simulink model "gnc_LocalAvoidance"  (R2026b)
settings: Solver=VariableStepAuto
values from neighbouring files (symbols this model uses):
  D = min(D, hypot(X - px(q) - t*ux, Y - py(q) - t*uy))    [gnc_globalReplanner.m]    (also in gnc_mpcPlantUpdate.m = zeros(2, 5))
  Ts = prm.Ts    [gnc_missionFSM.m]    (also in gnc_mpcPlantUpdate.m)
undefined symbols (not defined in the file or in its folder): P
libraries: simulink x3, navlib x1, robotalgslib x1
settings Model: Creator=aomar  LastModifiedBy=aomar

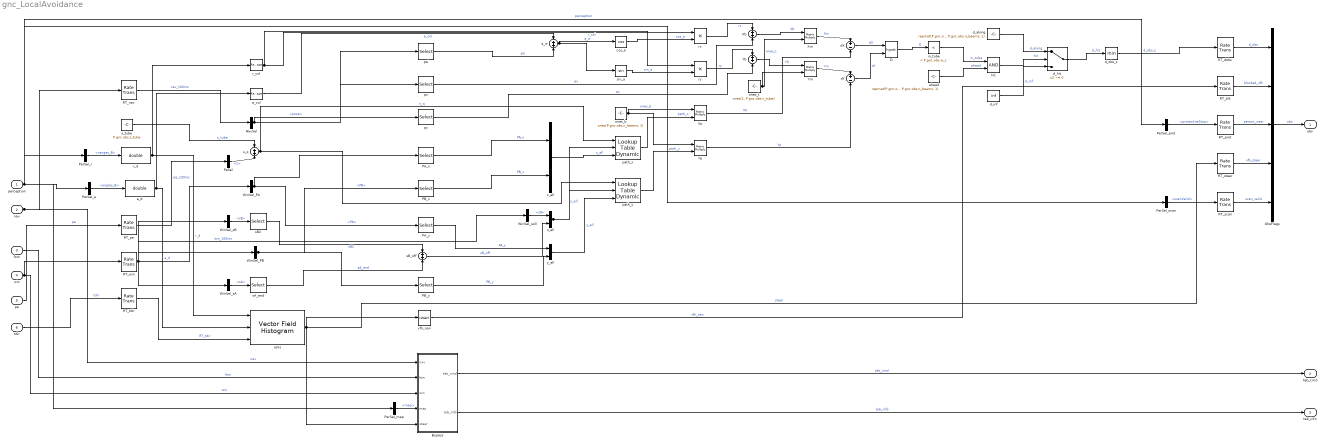
== system gnc_LocalAvoidance ==
  perception : Inport  OutDataTypeStr=Bus: Bus_Perception  SampleTime=Ts.perception
  nav : Inport  Port=2  OutDataTypeStr=Bus: Bus_NavCond  SampleTime=Ts.gnc
  fsm : Inport  Port=3  OutDataTypeStr=Bus: Bus_FsmOut  SampleTime=Ts.gnc
  win : Inport  Port=4  OutDataTypeStr=Bus: Bus_PathWindow  SampleTime=Ts.gnc
  pe : Inport  Port=5  OutDataTypeStr=Bus: Bus_PathError  SampleTime=Ts.gnc
  tdir : Inport  Port=6  OutDataTypeStr=double  PortDimensions=1  SampleTime=Ts.gnc
  Bypass : Subsystem  Variant=on
  D : Math  Operator=hypot
  NavSel : BusSelector  OutputSignals=pose
  ObsFlags : BusCreator  Inputs=5  OutDataTypeStr=Bus: Bus_ObsFlags  NonVirtualBus=on
  PA_x : Selector  NumberOfDimensions=2  InputPortWidth=3  IndexOptions=Select all,Index vector (dialog)  Indices=,1  OutputSizes=1
  PA_y : Selector  NumberOfDimensions=2  InputPortWidth=3  IndexOptions=Select all,Index vector (dialog)  Indices=,2  OutputSizes=1
  PB_x : Selector  NumberOfDimensions=2  InputPortWidth=3  IndexOptions=Index vector (dialog),Index vector (dialog)  Indices=2:P.gnc.path.N_smooth,1  OutputSizes=1
  PB_y : Selector  NumberOfDimensions=2  InputPortWidth=3  IndexOptions=Index vector (dialog),Index vector (dialog)  Indices=2:P.gnc.path.N_smooth,2  OutputSizes=1
  PeSel : BusSelector  OutputSignals=s
  PerSel_a : BusSelector  OutputSignals=angles_B
  PerSel_map : BusSelector  OutputSignals=map
  PerSel_prot : BusSelector  OutputSignals=protectiveStop
  PerSel_r : BusSelector  OutputSignals=ranges_B
  PerSel_scan : BusSelector  OutputSignals=scanValid
  RT_blk : RateTransition  OutPortSampleTime=Ts.gnc
  RT_dobs : RateTransition  InitialCondition=1e6  OutPortSampleTime=Ts.gnc
  RT_nav : RateTransition  OutPortSampleTime=Ts.gnc_avoid
  RT_pe : RateTransition  OutPortSampleTime=Ts.gnc_avoid
  RT_prot : RateTransition  OutPortSampleTime=Ts.gnc
  RT_scan : RateTransition  InitialCondition=false  OutPortSampleTime=Ts.gnc
  RT_steer : RateTransition  OutPortSampleTime=Ts.gnc
  RT_tdir : RateTransition  OutPortSampleTime=Ts.gnc_avoid
  RT_win : RateTransition  OutPortSampleTime=Ts.gnc_avoid
  VFH : robotalgslib/Vector Field Histogram  NumAngularSectors=P.gnc.vfh.NumAngularSectors  DistanceLimits=P.gnc.vfh.DistanceLimits  HistogramThresholds=P.gnc.vfh.HistogramThresholds  RobotRadius=P.gnc.vfh.RobotRadius  SafetyDistance=P.gnc.vfh.SafetyDistance  MinTurningRadius=P.gnc.vfh.MinTurningRadius  SimulateUsing=Code generation  TargetDirectionWeight=P.gnc.vfh.TargetDirectionWeight  CurrentDirectionWeight=P.gnc.vfh.CurrentDirectionWeight  PreviousDirectionWeight=P.gnc.vfh.PreviousDirectionWeight
      settings: LibrarySourceBlock=navlib/Control Algorithms/Vector Field Histogram
  WinSel_PA : BusSelector  OutputSignals=PA
  WinSel_PB : BusSelector  OutputSignals=PB
  WinSel_sA : BusSelector  OutputSignals=sA
  WinSel_sAll : BusSelector  OutputSignals=sA
  WinSel_sB : BusSelector  OutputSignals=sB
  Xb : Sum
  Xm : Product  Inputs=**  Multiplication=Matrix(*)
  Xp : Product  Inputs=**  Multiplication=Matrix(*)
  Yb : Sum
  Ym : Product  Inputs=**  Multiplication=Matrix(*)
  Yp : Product  Inputs=**  Multiplication=Matrix(*)
  a_col : Reshape  OutputDimensionality=Column vector (2-D)
  a_d : DataTypeConversion  OutDataTypeStr=double  RndMeth=Nearest
  a_w : Sum
  ahead : Constant  Value=repmat(P.gnc.obs.s_tube > P.gnc.obs.x_f, P.gnc.obs.n_beams, 1)  OutDataTypeStr=boolean  SampleTime=Ts.gnc_avoid
  cos_a : Trigonometry  Operator=cos
  dX : Sum  Inputs=+-
  dY : Sum  Inputs=+-
  d_along : Constant  Value=repmat(P.gnc.obs.s_tube - P.gnc.obs.x_f, P.gnc.obs.n_beams, 1)  OutDataTypeStr=double  SampleTime=Ts.gnc_avoid
  d_hit : Switch  Criteria=u2 ~= 0  SaturateOnIntegerOverflow=off  InputSameDT=off
  d_inf : Constant  Value=inf  OutDataTypeStr=double  SampleTime=Ts.gnc_avoid
  d_obs_s : MinMax
  hit : Logic  AllPortsSameDT=off  OutDataTypeStr=boolean
  in_tube : simulink/Logic and Bit Operations/Compare To Constant  relop=<  const=P.gnc.obs.w_c  OutDataTypeStr=boolean
  ones_b : Constant  Value=ones(P.gnc.obs.n_beams, 1)  VectorParams1D=off  OutDataTypeStr=double  SampleTime=Ts.gnc_avoid
  ones_t : Constant  Value=ones(1, P.gnc.obs.n_tube)  VectorParams1D=off  OutDataTypeStr=double  SampleTime=Ts.gnc_avoid
  path_x : simulink/Lookup Tables/Lookup Table Dynamic  LookUpMeth=Interpolation-Use End Values  OutDataType=fixdt('double')  OutScaling=2^-10  OutputDataTypeScalingMode=Specify via dialog  OutDataTypeStr=double  DoSatur=off
  path_y : simulink/Lookup Tables/Lookup Table Dynamic  LookUpMeth=Interpolation-Use End Values  OutDataType=fixdt('double')  OutScaling=2^-10  OutputDataTypeScalingMode=Specify via dialog  OutDataTypeStr=double  DoSatur=off
  psi : Selector  IndexOptions=Index vector (dialog)  Indices=3  OutputSizes=1
  px : Selector  IndexOptions=Index vector (dialog)  Indices=1  OutputSizes=1
  py : Selector  IndexOptions=Index vector (dialog)  Indices=2  OutputSizes=1
  r_col : Reshape  OutputDimensionality=Column vector (2-D)
  r_d : DataTypeConversion  OutDataTypeStr=double  RndMeth=Nearest
  rx : Product  Inputs=**
  ry : Product  Inputs=**
  sA_end : Selector  IndexOptions=Index vector (dialog)  Indices=P.gnc.path.N_smooth  OutputSizes=1
  sB2 : Selector  IndexOptions=Index vector (dialog)  Indices=2:P.gnc.path.N_smooth  OutputSizes=1
  sB_off : Sum
  s_all : Concatenate
  s_q : Sum
  s_tube : Constant  Value=P.gnc.obs.s_tube  VectorParams1D=off  OutDataTypeStr=double  SampleTime=Ts.gnc_avoid
  sin_a : Trigonometry
  vfh_nan : RelationalOperator  Operator=isNaN  OutDataTypeStr=boolean  RndMeth=Simplest  InputSameDT=off
  x_all : Concatenate
  y_all : Concatenate
  obs : Outport  OutDataTypeStr=Bus: Bus_ObsFlags
  teb_cmd : Outport  Port=2  OutDataTypeStr=double
  teb_info : Outport  Port=3  OutDataTypeStr=double
  wires:
  perception/1 -> PerSel_map/1, PerSel_prot/1, PerSel_r/1, PerSel_scan/1, PerSel_a/1  "perception"
  nav/1 -> Bypass/1(nav), RT_nav/1  "nav"
  fsm/1 -> Bypass/2(fsm)  "fsm"
  win/1 -> Bypass/3(win), RT_win/1  "win"
  pe/1 -> RT_pe/1  "pe"
  tdir/1 -> RT_tdir/1  "tdir"
  PerSel_r/1 -> r_d/1  "<ranges_B>"
  PerSel_a/1 -> a_d/1  "<angles_B>"
  s_tube/1 -> s_q/1  "s_tube"
  RT_nav/1 -> NavSel/1  "nav_100ms"
  RT_pe/1 -> PeSel/1  "pe_100ms"
  RT_win/1 -> WinSel_PA/1, WinSel_sAll/1, WinSel_sB/1, WinSel_sA/1, WinSel_PB/1  "win_100ms"
  RT_tdir/1 -> VFH/3  "RT_tdir"
  r_d/1 -> VFH/1, r_col/1  "r_d"
  a_d/1 -> VFH/2, a_col/1  "a_d"
  PeSel/1 -> s_q/2  "<s>"
  WinSel_sB/1 -> sB2/1  "<sB>"
  WinSel_sA/1 -> sA_end/1  "<sA>"
  NavSel/1 -> psi/1, px/1, py/1  "<pose>"
  WinSel_PA/1 -> PA_y/1, PA_x/1  "<PA>"
  WinSel_PB/1 -> PB_x/1, PB_y/1  "<PB>"
  s_q/1 -> path_y/1, path_x/1  "s_q"
  r_col/1 -> rx/1, ry/1  "r_col"
  a_col/1 -> a_w/1  "a_col"
  sB2/1 -> sB_off/1  "sB2"
  sA_end/1 -> sB_off/2  "sA_end"
  VFH/1 -> RT_steer/1, Bypass/5(steer), vfh_nan/1  "steer"
  PerSel_map/1 -> Bypass/4(map)  "<map>"
  sB_off/1 -> s_all/2  "sB_off"
  vfh_nan/1 -> RT_blk/1  "vfh_nan"
  psi/1 -> a_w/2  "psi"
  py/1 -> Yb/2  "py"
  PA_x/1 -> x_all/1  "PA_x"
  PB_x/1 -> x_all/2  "PB_x"
  PA_y/1 -> y_all/1  "PA_y"
  PB_y/1 -> y_all/2  "PB_y"
  Bypass/1(teb_cmd) -> teb_cmd/1  "teb_cmd"
  Bypass/2(teb_info) -> teb_info/1  "teb_info"
  WinSel_sAll/1 -> s_all/1  "<sA>"
  x_all/1 -> path_x/3  "x_all"
  s_all/1 -> path_x/2, path_y/2  "s_all"
  y_all/1 -> path_y/3  "y_all"
  a_w/1 -> sin_a/1, cos_a/1  "a_w"
  cos_a/1 -> rx/2  "cos_a"
  sin_a/1 -> ry/2  "sin_a"
  ones_b/1 -> Yp/1, Xp/1  "ones_b"
  path_x/1 -> Xp/2  "path_x"
  path_y/1 -> Yp/2  "path_y"
  rx/1 -> Xb/1  "rx"
  Xp/1 -> dX/2  "Xp"
  Yp/1 -> dY/2  "Yp"
  Xb/1 -> Xm/1  "Xb"
  Yb/1 -> Ym/1  "Yb"
  ones_t/1 -> Xm/2, Ym/2  "ones_t"
  Xm/1 -> dX/1  "Xm"
  Ym/1 -> dY/1  "Ym"
  dX/1 -> D/1  "dX"
  dY/1 -> D/2  "dY"
  D/1 -> in_tube/1  "D"
  in_tube/1 -> hit/1  "in_tube"
  ahead/1 -> hit/2  "ahead"
  d_along/1 -> d_hit/1  "d_along"
  hit/1 -> d_hit/2  "hit"
  d_inf/1 -> d_hit/3  "d_inf"
  d_hit/1 -> d_obs_s/1  "d_hit"
  d_obs_s/1 -> RT_dobs/1  "d_obs_s"
  PerSel_prot/1 -> RT_prot/1  "<protectiveStop>"
  PerSel_scan/1 -> RT_scan/1  "<scanValid>"
  RT_dobs/1 -> ObsFlags/1  "d_obs"
  RT_blk/1 -> ObsFlags/2  "blocked_vfh"
  RT_prot/1 -> ObsFlags/3  "person_near"
  RT_steer/1 -> ObsFlags/4  "vfh_steer"
  RT_scan/1 -> ObsFlags/5  "scan_valid"
  ObsFlags/1 -> obs/1  "obs"
  px/1 -> Xb/2  "px"
  ry/1 -> Yb/1  "ry"

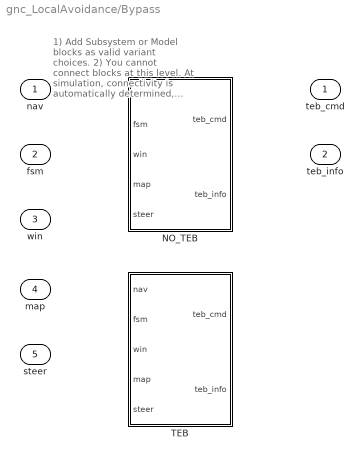
== system gnc_LocalAvoidance/Bypass ==
  note: 1) Add Subsystem or Model blocks as valid variant choices.
      | 2) You cannot connect blocks at this level. At simulation, connectivity is automatically
      | determined, based on the active variant and port name matching.
  nav : Inport
  fsm : Inport  Port=2
  win : Inport  Port=3
  map : Inport  Port=4
  steer : Inport  Port=5
  NO_TEB : Subsystem  VariantControl=VC_TEB == 0
  TEB : Subsystem  VariantControl=VC_TEB == 1
  teb_cmd : Outport
  teb_info : Outport  Port=2

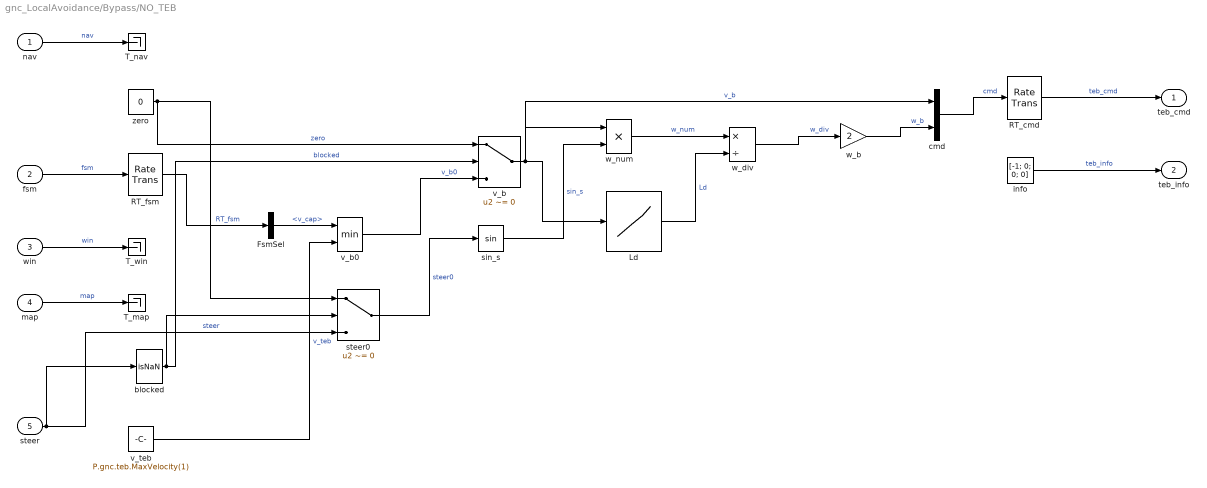
== system gnc_LocalAvoidance/Bypass/NO_TEB ==
  nav : Inport
  fsm : Inport  Port=2
  win : Inport  Port=3
  map : Inport  Port=4
  steer : Inport  Port=5
  FsmSel : BusSelector  OutputSignals=v_cap
  Ld : Lookup_n-D  NumberOfTableDimensions=1  BreakpointsForDimension1=P.gnc.obs.vfh_Ld_v  Table=P.gnc.obs.vfh_Ld  ExtrapMethod=Clip  UseLastTableValue=on  InternalRulePriority=Speed  RndMeth=Simplest
  RT_cmd : RateTransition  OutPortSampleTime=Ts.gnc
  RT_fsm : RateTransition  OutPortSampleTime=Ts.gnc_avoid
  T_map : Terminator
  T_nav : Terminator
  T_win : Terminator
  blocked : RelationalOperator  Operator=isNaN  OutDataTypeStr=boolean  RndMeth=Simplest  InputSameDT=off
  cmd : Mux  Inputs=2
  info : Constant  Value=[-1; 0; 0; 0]  OutDataTypeStr=double  SampleTime=Ts.gnc
  sin_s : Trigonometry
  steer0 : Switch  Criteria=u2 ~= 0  SaturateOnIntegerOverflow=off  InputSameDT=off
  v_b : Switch  Criteria=u2 ~= 0  SaturateOnIntegerOverflow=off  InputSameDT=off
  v_b0 : MinMax  Inputs=2
  v_teb : Constant  Value=P.gnc.teb.MaxVelocity(1)  OutDataTypeStr=double  SampleTime=Ts.gnc_avoid
  w_b : Gain  Gain=2
  w_div : Product  Inputs=*/
  w_num : Product  Inputs=**
  zero : Constant  Value=0  OutDataTypeStr=double  SampleTime=Ts.gnc_avoid
  teb_cmd : Outport
  teb_info : Outport  Port=2
  wires:
  nav/1 -> T_nav/1  "nav"
  fsm/1 -> RT_fsm/1  "fsm"
  win/1 -> T_win/1  "win"
  map/1 -> T_map/1  "map"
  steer/1 -> steer0/3, blocked/1  "steer"
  zero/1 -> steer0/1, v_b/1  "zero"
  v_teb/1 -> v_b0/2  "v_teb"
  RT_fsm/1 -> FsmSel/1  "RT_fsm"
  blocked/1 -> v_b/2, steer0/2  "blocked"
  FsmSel/1 -> v_b0/1  "<v_cap>"
  v_b0/1 -> v_b/3  "v_b0"
  steer0/1 -> sin_s/1  "steer0"
  sin_s/1 -> w_num/2  "sin_s"
  v_b/1 -> Ld/1, cmd/1, w_num/1  "v_b"
  w_num/1 -> w_div/1  "w_num"
  Ld/1 -> w_div/2  "Ld"
  w_div/1 -> w_b/1  "w_div"
  w_b/1 -> cmd/2  "w_b"
  cmd/1 -> RT_cmd/1  "cmd"
  info/1 -> teb_info/1  "teb_info"
  RT_cmd/1 -> teb_cmd/1  "teb_cmd"

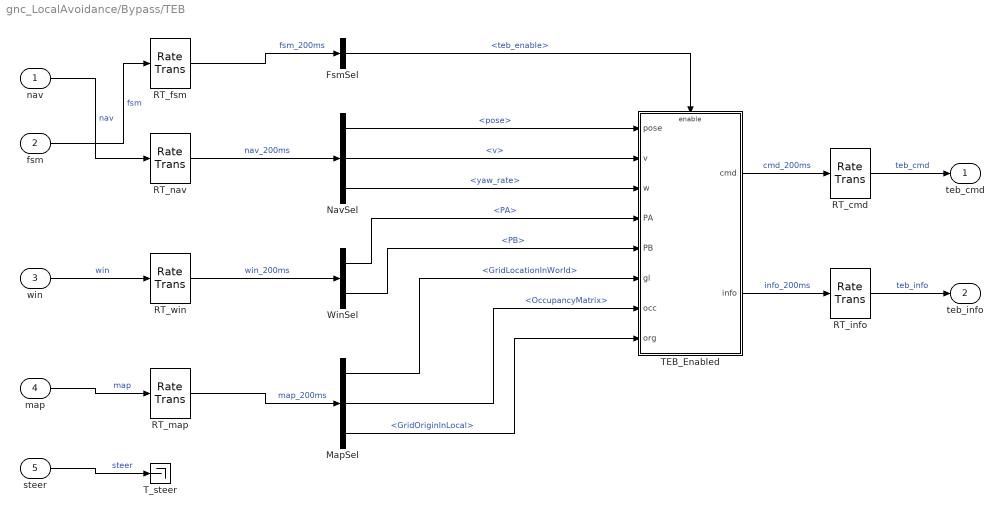
== system gnc_LocalAvoidance/Bypass/TEB ==
  nav : Inport
  fsm : Inport  Port=2
  win : Inport  Port=3
  map : Inport  Port=4
  steer : Inport  Port=5
  FsmSel : BusSelector  OutputSignals=teb_enable
  MapSel : BusSelector  OutputSignals=GridLocationInWorld,OccupancyMatrix,GridOriginInLocal
  NavSel : BusSelector  OutputSignals=pose,v,yaw_rate
  RT_cmd : RateTransition  OutPortSampleTime=Ts.gnc
  RT_fsm : RateTransition  OutPortSampleTime=P.gnc.teb.Ts
  RT_info : RateTransition  OutPortSampleTime=Ts.gnc
  RT_map : RateTransition  OutPortSampleTime=P.gnc.teb.Ts
  RT_nav : RateTransition  OutPortSampleTime=P.gnc.teb.Ts
  RT_win : RateTransition  OutPortSampleTime=P.gnc.teb.Ts
  TEB_Enabled : Subsystem  TreatAsAtomicUnit=on
  T_steer : Terminator
  WinSel : BusSelector  OutputSignals=PA,PB
  teb_cmd : Outport
  teb_info : Outport  Port=2
  wires:
  nav/1 -> RT_nav/1  "nav"
  fsm/1 -> RT_fsm/1  "fsm"
  win/1 -> RT_win/1  "win"
  map/1 -> RT_map/1  "map"
  steer/1 -> T_steer/1  "steer"
  RT_fsm/1 -> FsmSel/1  "fsm_200ms"
  RT_nav/1 -> NavSel/1  "nav_200ms"
  RT_win/1 -> WinSel/1  "win_200ms"
  RT_map/1 -> MapSel/1  "map_200ms"
  FsmSel/1 -> TEB_Enabled/Enable  "<teb_enable>"
  NavSel/1 -> TEB_Enabled/1(pose)  "<pose>"
  NavSel/2 -> TEB_Enabled/2(v)  "<v>"
  NavSel/3 -> TEB_Enabled/3(w)  "<yaw_rate>"
  WinSel/1 -> TEB_Enabled/4(PA)  "<PA>"
  WinSel/2 -> TEB_Enabled/5(PB)  "<PB>"
  MapSel/1 -> TEB_Enabled/6(gl)  "<GridLocationInWorld>"
  MapSel/2 -> TEB_Enabled/7(occ)  "<OccupancyMatrix>"
  MapSel/3 -> TEB_Enabled/8(org)  "<GridOriginInLocal>"
  TEB_Enabled/1(cmd) -> RT_cmd/1  "cmd_200ms"
  TEB_Enabled/2(info) -> RT_info/1  "info_200ms"
  RT_cmd/1 -> teb_cmd/1  "teb_cmd"
  RT_info/1 -> teb_info/1  "teb_info"

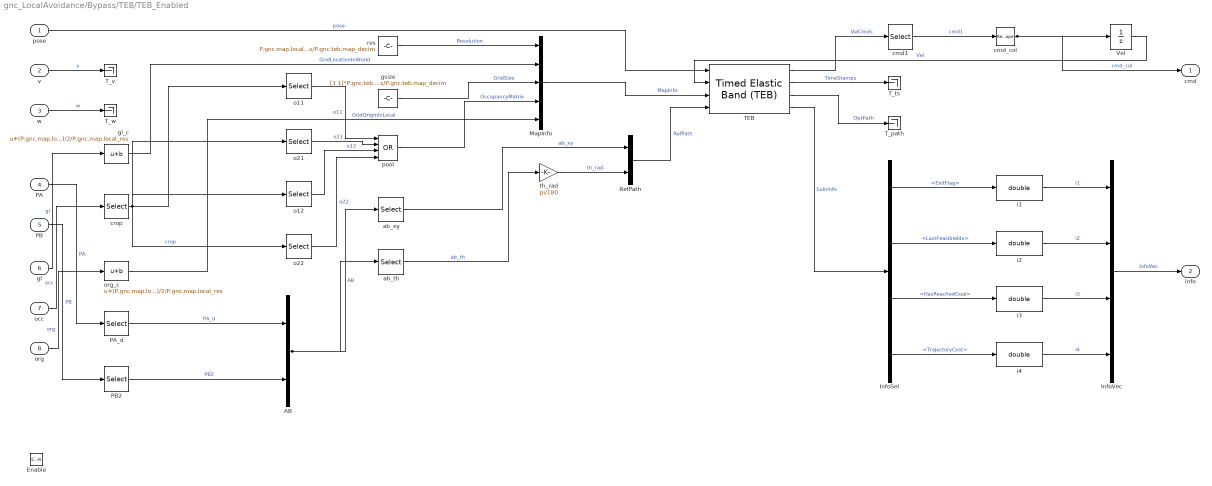
== system gnc_LocalAvoidance/Bypass/TEB/TEB_Enabled ==
  pose : Inport
  v : Inport  Port=2
  w : Inport  Port=3
  PA : Inport  Port=4
  PB : Inport  Port=5
  gl : Inport  Port=6
  occ : Inport  Port=7
  org : Inport  Port=8
  Enable : EnablePort  StatesWhenEnabling=reset  PropagateVarSize=During execution
  AB : Concatenate  Mode=Multidimensional array
  InfoSel : BusSelector  OutputSignals=ExitFlag,LastFeasibleIdx,HasReachedGoal,TrajectoryCost
  InfoVec : Mux
  MapInfo : BusCreator  Inputs=5  OutDataTypeStr=Bus: Bus_TebMapCrop  NonVirtualBus=on
  PA_d : Selector  NumberOfDimensions=2  InputPortWidth=3  IndexOptions=Index vector (dialog),Select all  Indices=1:P.gnc.teb.ref_decim:P.gnc.path.N_smooth,  OutputSizes=1
  PB2 : Selector  NumberOfDimensions=2  InputPortWidth=3  IndexOptions=Index vector (dialog),Select all  Indices=1 + P.gnc.teb.ref_decim:P.gnc.teb.ref_decim:P.gnc.path.N_smooth,  OutputSizes=1
  RefPath : Concatenate  Mode=Multidimensional array  ConcatenateDimension=2
  TEB : navlib/Control Algorithms/Timed Elastic Band (TEB)  ControlMode=Path Following with Obstacle Avoidance  SampleTime=-1  LookAheadTimePort=off  LookAheadTime=P.gnc.teb.LookAheadTime  GoalTolerancePort=off  GoalTolerance=P.gnc.teb.GoalTolerance  MaxVelocityPort=off  MaxVelocity=P.gnc.teb.MaxVelocity  MaxReverseVelocityPort=off  MaxReverseVelocity=NaN  MaxAccelerationPort=off  MaxAcceleration=P.gnc.teb.MaxAcceleration  MinTurningRadiusPort=off  MinTurningRadius=P.gnc.teb.MinTurningRadius  ReferenceDeltaTimePort=off  ReferenceDeltaTime=P.gnc.teb.ReferenceDeltaTime  NumIterationPort=off  NumIteration=P.gnc.teb.NumIteration  TimePort=off  Time=P.gnc.teb.Time  SmoothnessPort=off  Smoothness=P.gnc.teb.Smoothness  ObstaclePort=off  Obstacle=P.gnc.teb.Obstacle  Shape=Rectangle  Dimension=P.gnc.teb.Dimension  FixedTransform=se2  ObstacleSafetyMarginPort=off  ObstacleSafetyMargin=P.gnc.teb.ObstacleSafetyMargin
  T_path : Terminator
  T_ts : Terminator
  T_v : Terminator
  T_w : Terminator
  Vel : UnitDelay  InitialCondition=zeros(2,1)  SampleTime=-1
  ab_th : Selector  NumberOfDimensions=2  InputPortWidth=3  IndexOptions=Select all,Index vector (dialog)  Indices=,3  OutputSizes=1
  ab_xy : Selector  NumberOfDimensions=2  InputPortWidth=3  IndexOptions=Select all,Index vector (dialog)  Indices=,[1 2]  OutputSizes=1
  cmd1 : Selector  NumberOfDimensions=2  InputPortWidth=3  IndexOptions=Index vector (dialog),Index vector (dialog)  Indices=1,[1 2]  OutputSizes=1
  cmd_col : Reshape
  crop : Selector  NumberOfDimensions=2  InputPortWidth=3  IndexOptions=Index vector (dialog),Index vector (dialog)  Indices=(P.gnc.map.local_N - P.gnc.teb.map_window*P.gnc.map.local_res)/2 + (1:P.gnc.teb.map_window*P.gnc.map.local_res),(P.gnc.map.local_N - P.gnc.teb.map_window*P.gnc.map.local_res)/2 + (1:P.gnc.teb.map_window*P.gnc.map.local_res)  OutputSizes=1
  gl_c : Bias  Bias=(P.gnc.map.local_N - P.gnc.teb.map_window*P.gnc.map.local_res)/2/P.gnc.map.local_res  SaturateOnIntegerOverflow=off
  gsize : Constant  Value=[1 1]*P.gnc.teb.map_window*P.gnc.map.local_res/P.gnc.teb.map_decim  VectorParams1D=off  OutDataTypeStr=double  SampleTime=-1
  i{1..4} (4 alike) : DataTypeConversion  OutDataTypeStr=double  RndMeth=Nearest
  o11 : Selector  NumberOfDimensions=2  InputPortWidth=3  IndexOptions=Index vector (dialog),Index vector (dialog)  Indices=1:2:P.gnc.teb.map_window*P.gnc.map.local_res,1:2:P.gnc.teb.map_window*P.gnc.map.local_res  OutputSizes=1
  o12 : Selector  NumberOfDimensions=2  InputPortWidth=3  IndexOptions=Index vector (dialog),Index vector (dialog)  Indices=1:2:P.gnc.teb.map_window*P.gnc.map.local_res,2:2:P.gnc.teb.map_window*P.gnc.map.local_res  OutputSizes=1
  o21 : Selector  NumberOfDimensions=2  InputPortWidth=3  IndexOptions=Index vector (dialog),Index vector (dialog)  Indices=2:2:P.gnc.teb.map_window*P.gnc.map.local_res,1:2:P.gnc.teb.map_window*P.gnc.map.local_res  OutputSizes=1
  o22 : Selector  NumberOfDimensions=2  InputPortWidth=3  IndexOptions=Index vector (dialog),Index vector (dialog)  Indices=2:2:P.gnc.teb.map_window*P.gnc.map.local_res,2:2:P.gnc.teb.map_window*P.gnc.map.local_res  OutputSizes=1
  org_c : Bias  Bias=(P.gnc.map.local_N - P.gnc.teb.map_window*P.gnc.map.local_res)/2/P.gnc.map.local_res  SaturateOnIntegerOverflow=off
  pool : Logic  Operator=OR  Inputs=4  AllPortsSameDT=off  OutDataTypeStr=boolean
  res : Constant  Value=P.gnc.map.local_res/P.gnc.teb.map_decim  OutDataTypeStr=double  SampleTime=-1
  th_rad : Gain  Gain=pi/180
  cmd : Outport  OutputWhenDisabled=reset  InitialOutput=zeros(2,1)
  info : Outport  Port=2  OutputWhenDisabled=reset  InitialOutput=zeros(4,1)
  wires:
  pose/1 -> TEB/1  "pose"
  v/1 -> T_v/1  "v"
  w/1 -> T_w/1  "w"
  PA/1 -> PA_d/1  "PA"
  PB/1 -> PB2/1  "PB"
  gl/1 -> gl_c/1  "gl"
  occ/1 -> crop/1  "occ"
  org/1 -> org_c/1  "org"
  gl_c/1 -> MapInfo/2  "GridLocationInWorld"
  crop/1 -> o11/1, o21/1, o22/1, o12/1  "crop"
  org_c/1 -> MapInfo/5  "GridOriginInLocal"
  PA_d/1 -> AB/1  "PA_d"
  PB2/1 -> AB/2  "PB2"
  AB/1 -> ab_xy/1, ab_th/1  "AB"
  o11/1 -> pool/1  "o11"
  o21/1 -> pool/2  "o21"
  o12/1 -> pool/3  "o12"
  o22/1 -> pool/4  "o22"
  res/1 -> MapInfo/1  "Resolution"
  gsize/1 -> MapInfo/3  "GridSize"
  pool/1 -> MapInfo/4  "OccupancyMatrix"
  ab_xy/1 -> RefPath/1  "ab_xy"
  ab_th/1 -> th_rad/1  "ab_th"
  MapInfo/1 -> TEB/3  "MapInfo"
  th_rad/1 -> RefPath/2  "th_rad"
  RefPath/1 -> TEB/4  "RefPath"
  TEB/1 -> cmd1/1  "VelCmds"
  TEB/2 -> T_ts/1  "TimeStamps"
  TEB/3 -> T_path/1  "OptPath"
  TEB/4 -> InfoSel/1  "SolnInfo"
  InfoSel/1 -> i1/1  "<ExitFlag>"
  InfoSel/2 -> i2/1  "<LastFeasibleIdx>"
  InfoSel/3 -> i3/1  "<HasReachedGoal>"
  InfoSel/4 -> i4/1  "<TrajectoryCost>"
  cmd1/1 -> cmd_col/1  "cmd1"
  cmd_col/1 -> cmd/1, Vel/1  "cmd_col"
  i1/1 -> InfoVec/1  "i1"
  i2/1 -> InfoVec/2  "i2"
  i3/1 -> InfoVec/3  "i3"
  i4/1 -> InfoVec/4  "i4"
  InfoVec/1 -> info/1  "InfoVec"
  Vel/1 -> TEB/2  "Vel"
